simulink model "dual_thyristor_bridge_rectifier"  (R2025b)
settings: Solver=ode1be  StartTime=0.0  StopTime=simlength  FixedStep=tc  MaxStep=tc
values from neighbouring files (symbols this model uses):
  n1 = 35    [voltage_spectrum_analysis.m]
  omega_grid_emulator_nom = w_grid    (= 314.159265359)    [grid_emulator.m]
  vn_eta_pu = 0    [grid_emulator.m]
  vn_xi_pu = 0    [grid_emulator.m]
  vp_xi_pu = 1    [grid_emulator.m]
  w_grid = f_grid*2*pi    (= 314.159265359)    [grid_emulator.m]
undefined symbols (not defined in the file or in its folder): CSF_11, CSF_13, CSF_5, CSF_7, delta_fht1, Idc_traction_normalization_factor, ki_u_ctrl, kp_u_ctrl, Ld_fht1, LFu_dc, LSF_11, LSF_13, LSF_5, LSF_7, magnitude, n10, omega_fht1, pll_i1, pll_p, RLFu_dc, tc, Tcontrol_rect, ts_ctrl_rect, ugrid_factor, Vdc_traction_normalization_factor, Vgrid_phase_normalization_factor
libraries: fl_lib x299, nesl_utility x67, ee_lib x24, single_phase_transformer_lib x3, cstblocks x3
(part 3 of 6)

== system dual_thyristor_bridge_rectifier/dual_rectifier_bridge/neg_bridge/firing2 ==
  Capacitor1 : fl_lib/Electrical/Electrical Elements/Capacitor  Commented=on  c=100e-6 F  r=1e-6 Ohm  g=0 1/Ohm  i_specify=off  i_priority=None  i=0 A  i_nominal_specify=off  i_nominal_value=1  i_nominal_unit=A  v_specify=off  v_priority=None  v=0 V  v_nominal_specify=off  v_nominal_value=1  v_nominal_unit=V  vc_specify=off  vc_priority=High  vc=0 V  vc_nominal_specify=off  vc_nominal_value=1  vc_nominal_unit=V
  Capacitor2 : fl_lib/Electrical/Electrical Elements/Capacitor  Commented=on  c=100e-12 F  r=1e-6 Ohm  g=0 1/Ohm  i_specify=off  i_priority=None  i=0 A  i_nominal_specify=off  i_nominal_value=1  i_nominal_unit=A  v_specify=off  v_priority=None  v=0 V  v_nominal_specify=off  v_nominal_value=1  v_nominal_unit=V  vc_specify=off  vc_priority=High  vc=0 V  vc_nominal_specify=off  vc_nominal_value=1  vc_nominal_unit=V
  Controlled Voltage Source1 : fl_lib/Electrical/Electrical Sources/Controlled Voltage Source  Commented=on
  Controlled Voltage Source2 : fl_lib/Electrical/Electrical Sources/Controlled Voltage Source  Commented=on
  Diode : fl_lib/Electrical/Electrical Elements/Diode  Commented=on  Vf=0.6 V  Ron=0.3 Ohm  Goff=1e-8 1/Ohm  i_specify=off  i_priority=None  i=0 A  i_nominal_specify=off  i_nominal_value=1  i_nominal_unit=A  v_specify=off  v_priority=None  v=0 V  v_nominal_specify=off  v_nominal_value=1  v_nominal_unit=V
  Diode2 : fl_lib/Electrical/Electrical Elements/Diode  Commented=on  Vf=0.6 V  Ron=0.3 Ohm  Goff=1e-8 1/Ohm  i_specify=off  i_priority=None  i=0 A  i_nominal_specify=off  i_nominal_value=1  i_nominal_unit=A  v_specify=off  v_priority=None  v=0 V  v_nominal_specify=off  v_nominal_value=1  v_nominal_unit=V
  Diode3 : fl_lib/Electrical/Electrical Elements/Diode  Commented=on  Vf=0.6 V  Ron=0.3 Ohm  Goff=1e-8 1/Ohm  i_specify=off  i_priority=None  i=0 A  i_nominal_specify=off  i_nominal_value=1  i_nominal_unit=A  v_specify=off  v_priority=None  v=0 V  v_nominal_specify=off  v_nominal_value=1  v_nominal_unit=V
  Electrical Reference3 : fl_lib/Electrical/Electrical Elements/Electrical Reference  Commented=on
  Electrical Reference4 : fl_lib/Electrical/Electrical Elements/Electrical Reference  Commented=on
  Electrical Reference5 : fl_lib/Electrical/Electrical Elements/Electrical Reference  Commented=on
  "IGBT (Ideal, Switching)" : ee_lib/Semiconductors & Converters/IGBT (Ideal, Switching)  Commented=on  port_option=ee.enum.controlport.elec  Vf=0.8 V  Ron=0.001 Ohm  Goff=1e-5 1/Ohm  Vth=2 V  diode_param=1  diode_Vf=0.8 V  diode_Ron=0.001 Ohm  diode_Goff=1e-5 1/Ohm  diode_C=50e-9 F  diode_iRM=-235 A  diode_iF=300 A  diode_idot=-50 A/us  diode_trr_param=1  diode_trr_factor=3  diode_trr=15 us  diode_Qrr=1500 s*uA  ice_specify=off  ice_priority=None  ice=0 A  ice_nominal_specify=off  ice_nominal_value=1  ice_nominal_unit=A  vce_specify=off  vce_priority=None  vce=0 V  vce_nominal_specify=off  vce_nominal_value=1  vce_nominal_unit=V  vge_specify=off  vge_priority=None  vge=0 V  vge_nominal_specify=off  vge_nominal_value=1  vge_nominal_unit=V  thermal_loss_option=2  Von_data=[0, 1.1, 1.3, 1.45, 1.75, 2.25, 2.7; 0, 1, 1.15, 1.35, 1.7, 2.35, 3] V  Tj=[298.15, 398.15] K  Iout_data=[0, 10, 50, 100, 200, 400, 600] A  Eon_data=[0, .29, 1.43, 2.86, 5.71, 13.14, 22.86; 0, .57, 2.63, 5.14, 10.29, 20.57, 30.29] * 1e-3 J  Eoff_data=[0, .21, 1.07, 2.14, 4.29, 9.86, 17.14; 0, .43, 1.97, 3.86, 7.71, 15.43, 22.71] * 1e-3 J  Eon_data_3D=[zeros(2, 9, 3)] J  Eoff_data_3D=[zeros(2, 9, 3)] J  Tj_loss=[298.15, 398.15] K  Iout_data_loss=[0, .1, 1, 5, 10, 20, 40, 70, 100] A  tabulateWithVce=false  Vce_loss=[0, 150, 300] V  Eon_scalar=22.86e-3 J  Eoff_scalar=17.14e-3 J  Voff=300 V  Iout_scalar=600 A  useCurrentFromPreviousCycle=false  useVoltageFromPreviousCycle=false  diodeModelType=ee.enum.converters.diodeModelType.pwl  diodeTableType=ee.enum.diode.tableType.IfMat  diode_ReverseIVType=ee.enum.diode.diodeReverseIV.constant  diode_IfMat=[.07, .12, .19, 1.75, 4.24, 7.32, 11.2; .16, .3, .72, 2.14, 4.02, 6.35, 9.12] A  diode_VfMat=[.9, 1.15, 1.25, 1.5, 1.75, 2.17, 2.6, 2.85; .58, .68, .75, 1.1, 1.38, 1.77, 2.27, 2.7] V  diode_TjVec=[25, 125] degC  diode_VfVec=[.5, .7, .9, 1.3, 1.7, 2.1, 2.5] V  diode_IfVec=[.1, .2, .5, 1, 2, 4, 7, 10] A  diode_IrMat=[1e-06, 2e-06, 5e-06, 1e-05, 2.5e-05, 5e-05, .0001; 2e-06, 5e-06, 1e-05, 4e-05, 8e-05, .0002, .0005] A  diode_VrMat=[10, 100, 200, 250, 300, 325, 350; 10, 70, 160, 220, 270, 300, 320] V  diode_VrVec=[10, 20, 40, 50, 70, 80, 100] V  diode_IrVec=[1e-06, 2e-06, 5e-06, 1e-05, 2e-05, 5e-05, .0001] A  diode_Vr=-600 V  diode_Ls=150 nH  diode_Erec=0.03 J  diode_rec_loss_model=ee.enum.diode.reverseRecoveryModel.fixed  diode_ErecVal=0 J  diode_scaleWithIandV=true  diode_ErecMat=zeros(2, 3) J  diode_TjrecVec=[298.15, 398.15] K  diode_IfrecVec=[.1, 1, 10] A  diode_IrecVal=10 A  diode_VrecVal=10 V  diode_tFilter=1 / 1000 / 100 s  separateThermalPortForDiode=false  thermal_network_parameterization=ee.enum.thermalNetworkTopology.external  Rth=[.08, .5] K/W  Rth_Cauer=[.08, .1, .5] K/W  Rth_Foster=[.08, .14, .22, .16] K/W  thermal_mass_parameterization=ee.enum.thermalNetwork.timeconstant  thermal_mass=[.01, .5] J/K  thermal_mass_Cauer=[.01, .1, .5] J/K  thermal_mass_Foster=[.001, .005, .05, .5] J/K  thermal_time_constant=[.001, .2] s  thermal_time_constant_Cauer=[.001, .1, .2] s  thermal_time_constant_Foster=[7e-05, .0007, .01, .08] s  thermal_mass_initial_temperatures=[25, 25] degC  thermal_mass_initial_temperatures_Cauer=[25, 25, 25] degC  junction_thermal_mass=0.01 J/K  Tvec_initial_Foster=[25, 25, 25, 25] degC  RthDiode=[.03, .2] K/W  RthCauerDiode=[.03, .1, .2] K/W  RthFosterDiode=[.03, .2] K/W  thermalMassDiode=[3, 25] J/K  thermalMassCauerDiode=[3, 10, 25] J/K  thermalMassFosterDiode=[33, 50] J/K  thermalTauDiode=[.1, 5] s  thermalTauCauerDiode=[.1, 1, 5] s  thermalTauFosterDiode=[1, 10] s  thermalMassInitTempDiode=[25, 25] degC  thermalMassInitTempCauerDiode=[25, 25, 25] degC  junctionthermalMassDiode=0.1 J/K  TVecInitialFosterDiode=[25, 25, 25, 25] degC  no_thermal_network=0  IGBT_junction_temperature_specify=off  IGBT_junction_temperature_priority=None  IGBT_junction_temperature=25 degC  IGBT_junction_temperature_nominal_specify=off  IGBT_junction_temperature_nominal_value=1  IGBT_junction_temperature_nominal_unit=degC  diode_junction_temperature_specify=off  diode_junction_temperature_priority=None  diode_junction_temperature=25 degC  diode_junction_temperature_nominal_specify=off  diode_junction_temperature_nominal_value=1  diode_junction_temperature_nominal_unit=degC  Qj_specify=off  Qj_priority=None  Qj=0 W  Qj_nominal_specify=off  Qj_nominal_value=1  Qj_nominal_unit=W  accumulatedSwitchingLosses_specify=off  accumulatedSwitchingLosses_priority=None  accumulatedSwitchingLosses=0 J
      settings: InternalSimscapePortConfiguration="{\"Bottom\":[],\"Left\":[{\"id\":\"G_elec\",\"label\":\"\",\"type\":\"foundation.electrical.electrical\"}],\"Right\":[{\"id\":\"C\",\"label\":\"\",\"type\":\"foundation.electrical.electrical\"},{\"id\":\"E\",\"label\":\"\",\"type\":\"foundation.electrical.electrical\"}],\"Top\":[]}"
  Ideal Transformer : fl_lib/Electrical/Electrical Elements/Ideal Transformer  Commented=on  n=2  i1_specify=off  i1_priority=None  i1=0 A  i1_nominal_specify=off  i1_nominal_value=1  i1_nominal_unit=A  v1_specify=off  v1_priority=None  v1=0 V  v1_nominal_specify=off  v1_nominal_value=1  v1_nominal_unit=V  i2_specify=off  i2_priority=None  i2=0 A  i2_nominal_specify=off  i2_nominal_value=1  i2_nominal_unit=A  v2_specify=off  v2_priority=None  v2=0 V  v2_nominal_specify=off  v2_nominal_value=1  v2_nominal_unit=V
  PS Constant : fl_lib/Physical Signals/Sources/PS Constant  Commented=on  constant=48 V
  Resistor1 : fl_lib/Electrical/Electrical Elements/Resistor  Commented=on  R=470 Ohm  i_specify=off  i_priority=None  i=0 A  i_nominal_specify=off  i_nominal_value=1  i_nominal_unit=A  v_specify=off  v_priority=None  v=0 V  v_nominal_specify=off  v_nominal_value=1  v_nominal_unit=V
  Resistor3 : fl_lib/Electrical/Electrical Elements/Resistor  Commented=on  R=470 Ohm  i_specify=off  i_priority=None  i=0 A  i_nominal_specify=off  i_nominal_value=1  i_nominal_unit=A  v_specify=off  v_priority=None  v=0 V  v_nominal_specify=off  v_nominal_value=1  v_nominal_unit=V
  Resistor5 : fl_lib/Electrical/Electrical Elements/Resistor  Commented=on  R=100 Ohm  i_specify=off  i_priority=None  i=0 A  i_nominal_specify=off  i_nominal_value=1  i_nominal_unit=A  v_specify=off  v_priority=None  v=0 V  v_nominal_specify=off  v_nominal_value=1  v_nominal_unit=V
  Resistor6 : fl_lib/Electrical/Electrical Elements/Resistor  Commented=on  R=1e9 Ohm  i_specify=off  i_priority=None  i=0 A  i_nominal_specify=off  i_nominal_value=1  i_nominal_unit=A  v_specify=off  v_priority=None  v=0 V  v_nominal_specify=off  v_nominal_value=1  v_nominal_unit=V
  Voltage Sensor : fl_lib/Electrical/Electrical Sensors/Voltage Sensor  Commented=on
  oscillator : Subsystem  Commented=on
  gin : PMIOPort  Side=Left
  g+ : PMIOPort  Port=2  Side=Right
  connections:
  "IGBT (Ideal, Switching)"/LConn1 -- Resistor1/RConn1
  Electrical Reference4/LConn1 -- Diode/LConn1 -- Ideal Transformer/LConn2
  Controlled Voltage Source2/LConn1 -- Resistor1/LConn1
  Controlled Voltage Source2/RConn2 -- Controlled Voltage Source1/RConn2 -- "IGBT (Ideal, Switching)"/RConn2 -- Ideal Transformer/LConn1 -- Diode/RConn1
  Ideal Transformer/RConn1 -- Diode2/LConn1
  Capacitor2/RConn1 -- Voltage Sensor/RConn2 -- Ideal Transformer/RConn2 -- Resistor6/LConn1 -- Resistor5/RConn1
  Diode2/RConn1 -- Resistor5/LConn1 -- Voltage Sensor/LConn1 -- Capacitor2/LConn1
  PS Constant/RConn1 -- Controlled Voltage Source1/RConn1
  Resistor6/RConn1 -- Electrical Reference3/LConn1
  "IGBT (Ideal, Switching)"/RConn1 -- Diode3/RConn1
  Diode3/LConn1 -- Resistor3/RConn1 -- Capacitor1/LConn1
  Electrical Reference5/LConn1 -- Capacitor1/RConn1
  Resistor3/LConn1 -- Controlled Voltage Source1/LConn1
  gin/RConn1 -- g+/RConn1

== system dual_thyristor_bridge_rectifier/dual_rectifier_bridge/neg_bridge/firing3 ==
  Capacitor1 : fl_lib/Electrical/Electrical Elements/Capacitor  Commented=on  c=100e-6 F  r=1e-6 Ohm  g=0 1/Ohm  i_specify=off  i_priority=None  i=0 A  i_nominal_specify=off  i_nominal_value=1  i_nominal_unit=A  v_specify=off  v_priority=None  v=0 V  v_nominal_specify=off  v_nominal_value=1  v_nominal_unit=V  vc_specify=off  vc_priority=High  vc=0 V  vc_nominal_specify=off  vc_nominal_value=1  vc_nominal_unit=V
  Capacitor2 : fl_lib/Electrical/Electrical Elements/Capacitor  Commented=on  c=100e-12 F  r=1e-6 Ohm  g=0 1/Ohm  i_specify=off  i_priority=None  i=0 A  i_nominal_specify=off  i_nominal_value=1  i_nominal_unit=A  v_specify=off  v_priority=None  v=0 V  v_nominal_specify=off  v_nominal_value=1  v_nominal_unit=V  vc_specify=off  vc_priority=High  vc=0 V  vc_nominal_specify=off  vc_nominal_value=1  vc_nominal_unit=V
  Controlled Voltage Source1 : fl_lib/Electrical/Electrical Sources/Controlled Voltage Source  Commented=on
  Controlled Voltage Source2 : fl_lib/Electrical/Electrical Sources/Controlled Voltage Source  Commented=on
  Diode : fl_lib/Electrical/Electrical Elements/Diode  Commented=on  Vf=0.6 V  Ron=0.3 Ohm  Goff=1e-8 1/Ohm  i_specify=off  i_priority=None  i=0 A  i_nominal_specify=off  i_nominal_value=1  i_nominal_unit=A  v_specify=off  v_priority=None  v=0 V  v_nominal_specify=off  v_nominal_value=1  v_nominal_unit=V
  Diode2 : fl_lib/Electrical/Electrical Elements/Diode  Commented=on  Vf=0.6 V  Ron=0.3 Ohm  Goff=1e-8 1/Ohm  i_specify=off  i_priority=None  i=0 A  i_nominal_specify=off  i_nominal_value=1  i_nominal_unit=A  v_specify=off  v_priority=None  v=0 V  v_nominal_specify=off  v_nominal_value=1  v_nominal_unit=V
  Diode3 : fl_lib/Electrical/Electrical Elements/Diode  Commented=on  Vf=0.6 V  Ron=0.3 Ohm  Goff=1e-8 1/Ohm  i_specify=off  i_priority=None  i=0 A  i_nominal_specify=off  i_nominal_value=1  i_nominal_unit=A  v_specify=off  v_priority=None  v=0 V  v_nominal_specify=off  v_nominal_value=1  v_nominal_unit=V
  Electrical Reference3 : fl_lib/Electrical/Electrical Elements/Electrical Reference  Commented=on
  Electrical Reference4 : fl_lib/Electrical/Electrical Elements/Electrical Reference  Commented=on
  Electrical Reference5 : fl_lib/Electrical/Electrical Elements/Electrical Reference  Commented=on
  "IGBT (Ideal, Switching)" : ee_lib/Semiconductors & Converters/IGBT (Ideal, Switching)  Commented=on  port_option=ee.enum.controlport.elec  Vf=0.8 V  Ron=0.001 Ohm  Goff=1e-5 1/Ohm  Vth=2 V  diode_param=1  diode_Vf=0.8 V  diode_Ron=0.001 Ohm  diode_Goff=1e-5 1/Ohm  diode_C=50e-9 F  diode_iRM=-235 A  diode_iF=300 A  diode_idot=-50 A/us  diode_trr_param=1  diode_trr_factor=3  diode_trr=15 us  diode_Qrr=1500 s*uA  ice_specify=off  ice_priority=None  ice=0 A  ice_nominal_specify=off  ice_nominal_value=1  ice_nominal_unit=A  vce_specify=off  vce_priority=None  vce=0 V  vce_nominal_specify=off  vce_nominal_value=1  vce_nominal_unit=V  vge_specify=off  vge_priority=None  vge=0 V  vge_nominal_specify=off  vge_nominal_value=1  vge_nominal_unit=V  thermal_loss_option=2  Von_data=[0, 1.1, 1.3, 1.45, 1.75, 2.25, 2.7; 0, 1, 1.15, 1.35, 1.7, 2.35, 3] V  Tj=[298.15, 398.15] K  Iout_data=[0, 10, 50, 100, 200, 400, 600] A  Eon_data=[0, .29, 1.43, 2.86, 5.71, 13.14, 22.86; 0, .57, 2.63, 5.14, 10.29, 20.57, 30.29] * 1e-3 J  Eoff_data=[0, .21, 1.07, 2.14, 4.29, 9.86, 17.14; 0, .43, 1.97, 3.86, 7.71, 15.43, 22.71] * 1e-3 J  Eon_data_3D=[zeros(2, 9, 3)] J  Eoff_data_3D=[zeros(2, 9, 3)] J  Tj_loss=[298.15, 398.15] K  Iout_data_loss=[0, .1, 1, 5, 10, 20, 40, 70, 100] A  tabulateWithVce=false  Vce_loss=[0, 150, 300] V  Eon_scalar=22.86e-3 J  Eoff_scalar=17.14e-3 J  Voff=300 V  Iout_scalar=600 A  useCurrentFromPreviousCycle=false  useVoltageFromPreviousCycle=false  diodeModelType=ee.enum.converters.diodeModelType.pwl  diodeTableType=ee.enum.diode.tableType.IfMat  diode_ReverseIVType=ee.enum.diode.diodeReverseIV.constant  diode_IfMat=[.07, .12, .19, 1.75, 4.24, 7.32, 11.2; .16, .3, .72, 2.14, 4.02, 6.35, 9.12] A  diode_VfMat=[.9, 1.15, 1.25, 1.5, 1.75, 2.17, 2.6, 2.85; .58, .68, .75, 1.1, 1.38, 1.77, 2.27, 2.7] V  diode_TjVec=[25, 125] degC  diode_VfVec=[.5, .7, .9, 1.3, 1.7, 2.1, 2.5] V  diode_IfVec=[.1, .2, .5, 1, 2, 4, 7, 10] A  diode_IrMat=[1e-06, 2e-06, 5e-06, 1e-05, 2.5e-05, 5e-05, .0001; 2e-06, 5e-06, 1e-05, 4e-05, 8e-05, .0002, .0005] A  diode_VrMat=[10, 100, 200, 250, 300, 325, 350; 10, 70, 160, 220, 270, 300, 320] V  diode_VrVec=[10, 20, 40, 50, 70, 80, 100] V  diode_IrVec=[1e-06, 2e-06, 5e-06, 1e-05, 2e-05, 5e-05, .0001] A  diode_Vr=-600 V  diode_Ls=150 nH  diode_Erec=0.03 J  diode_rec_loss_model=ee.enum.diode.reverseRecoveryModel.fixed  diode_ErecVal=0 J  diode_scaleWithIandV=true  diode_ErecMat=zeros(2, 3) J  diode_TjrecVec=[298.15, 398.15] K  diode_IfrecVec=[.1, 1, 10] A  diode_IrecVal=10 A  diode_VrecVal=10 V  diode_tFilter=1 / 1000 / 100 s  separateThermalPortForDiode=false  thermal_network_parameterization=ee.enum.thermalNetworkTopology.external  Rth=[.08, .5] K/W  Rth_Cauer=[.08, .1, .5] K/W  Rth_Foster=[.08, .14, .22, .16] K/W  thermal_mass_parameterization=ee.enum.thermalNetwork.timeconstant  thermal_mass=[.01, .5] J/K  thermal_mass_Cauer=[.01, .1, .5] J/K  thermal_mass_Foster=[.001, .005, .05, .5] J/K  thermal_time_constant=[.001, .2] s  thermal_time_constant_Cauer=[.001, .1, .2] s  thermal_time_constant_Foster=[7e-05, .0007, .01, .08] s  thermal_mass_initial_temperatures=[25, 25] degC  thermal_mass_initial_temperatures_Cauer=[25, 25, 25] degC  junction_thermal_mass=0.01 J/K  Tvec_initial_Foster=[25, 25, 25, 25] degC  RthDiode=[.03, .2] K/W  RthCauerDiode=[.03, .1, .2] K/W  RthFosterDiode=[.03, .2] K/W  thermalMassDiode=[3, 25] J/K  thermalMassCauerDiode=[3, 10, 25] J/K  thermalMassFosterDiode=[33, 50] J/K  thermalTauDiode=[.1, 5] s  thermalTauCauerDiode=[.1, 1, 5] s  thermalTauFosterDiode=[1, 10] s  thermalMassInitTempDiode=[25, 25] degC  thermalMassInitTempCauerDiode=[25, 25, 25] degC  junctionthermalMassDiode=0.1 J/K  TVecInitialFosterDiode=[25, 25, 25, 25] degC  no_thermal_network=0  IGBT_junction_temperature_specify=off  IGBT_junction_temperature_priority=None  IGBT_junction_temperature=25 degC  IGBT_junction_temperature_nominal_specify=off  IGBT_junction_temperature_nominal_value=1  IGBT_junction_temperature_nominal_unit=degC  diode_junction_temperature_specify=off  diode_junction_temperature_priority=None  diode_junction_temperature=25 degC  diode_junction_temperature_nominal_specify=off  diode_junction_temperature_nominal_value=1  diode_junction_temperature_nominal_unit=degC  Qj_specify=off  Qj_priority=None  Qj=0 W  Qj_nominal_specify=off  Qj_nominal_value=1  Qj_nominal_unit=W  accumulatedSwitchingLosses_specify=off  accumulatedSwitchingLosses_priority=None  accumulatedSwitchingLosses=0 J
      settings: InternalSimscapePortConfiguration="{\"Bottom\":[],\"Left\":[{\"id\":\"G_elec\",\"label\":\"\",\"type\":\"foundation.electrical.electrical\"}],\"Right\":[{\"id\":\"C\",\"label\":\"\",\"type\":\"foundation.electrical.electrical\"},{\"id\":\"E\",\"label\":\"\",\"type\":\"foundation.electrical.electrical\"}],\"Top\":[]}"
  Ideal Transformer : fl_lib/Electrical/Electrical Elements/Ideal Transformer  Commented=on  n=2  i1_specify=off  i1_priority=None  i1=0 A  i1_nominal_specify=off  i1_nominal_value=1  i1_nominal_unit=A  v1_specify=off  v1_priority=None  v1=0 V  v1_nominal_specify=off  v1_nominal_value=1  v1_nominal_unit=V  i2_specify=off  i2_priority=None  i2=0 A  i2_nominal_specify=off  i2_nominal_value=1  i2_nominal_unit=A  v2_specify=off  v2_priority=None  v2=0 V  v2_nominal_specify=off  v2_nominal_value=1  v2_nominal_unit=V
  PS Constant : fl_lib/Physical Signals/Sources/PS Constant  Commented=on  constant=48 V
  Resistor1 : fl_lib/Electrical/Electrical Elements/Resistor  Commented=on  R=470 Ohm  i_specify=off  i_priority=None  i=0 A  i_nominal_specify=off  i_nominal_value=1  i_nominal_unit=A  v_specify=off  v_priority=None  v=0 V  v_nominal_specify=off  v_nominal_value=1  v_nominal_unit=V
  Resistor3 : fl_lib/Electrical/Electrical Elements/Resistor  Commented=on  R=470 Ohm  i_specify=off  i_priority=None  i=0 A  i_nominal_specify=off  i_nominal_value=1  i_nominal_unit=A  v_specify=off  v_priority=None  v=0 V  v_nominal_specify=off  v_nominal_value=1  v_nominal_unit=V
  Resistor5 : fl_lib/Electrical/Electrical Elements/Resistor  Commented=on  R=100 Ohm  i_specify=off  i_priority=None  i=0 A  i_nominal_specify=off  i_nominal_value=1  i_nominal_unit=A  v_specify=off  v_priority=None  v=0 V  v_nominal_specify=off  v_nominal_value=1  v_nominal_unit=V
  Resistor6 : fl_lib/Electrical/Electrical Elements/Resistor  Commented=on  R=1e9 Ohm  i_specify=off  i_priority=None  i=0 A  i_nominal_specify=off  i_nominal_value=1  i_nominal_unit=A  v_specify=off  v_priority=None  v=0 V  v_nominal_specify=off  v_nominal_value=1  v_nominal_unit=V
  Voltage Sensor : fl_lib/Electrical/Electrical Sensors/Voltage Sensor  Commented=on
  oscillator : Subsystem  Commented=on
  gin : PMIOPort  Side=Left
  g+ : PMIOPort  Port=2  Side=Right
  connections:
  Resistor3/LConn1 -- Controlled Voltage Source1/LConn1
  Electrical Reference5/LConn1 -- Capacitor1/RConn1
  Capacitor1/LConn1 -- Resistor3/RConn1 -- Diode3/LConn1
  "IGBT (Ideal, Switching)"/RConn1 -- Diode3/RConn1
  Resistor6/RConn1 -- Electrical Reference3/LConn1
  PS Constant/RConn1 -- Controlled Voltage Source1/RConn1
  Capacitor2/LConn1 -- Voltage Sensor/LConn1 -- Resistor5/LConn1 -- Diode2/RConn1
  Resistor5/RConn1 -- Resistor6/LConn1 -- Ideal Transformer/RConn2 -- Voltage Sensor/RConn2 -- Capacitor2/RConn1
  Ideal Transformer/RConn1 -- Diode2/LConn1
  Diode/RConn1 -- Ideal Transformer/LConn1 -- "IGBT (Ideal, Switching)"/RConn2 -- Controlled Voltage Source1/RConn2 -- Controlled Voltage Source2/RConn2
  Controlled Voltage Source2/LConn1 -- Resistor1/LConn1
  Ideal Transformer/LConn2 -- Diode/LConn1 -- Electrical Reference4/LConn1
  "IGBT (Ideal, Switching)"/LConn1 -- Resistor1/RConn1
  gin/RConn1 -- g+/RConn1

== system dual_thyristor_bridge_rectifier/dual_rectifier_bridge/neg_bridge/firing4 ==
  Capacitor1 : fl_lib/Electrical/Electrical Elements/Capacitor  Commented=on  c=100e-6 F  r=1e-6 Ohm  g=0 1/Ohm  i_specify=off  i_priority=None  i=0 A  i_nominal_specify=off  i_nominal_value=1  i_nominal_unit=A  v_specify=off  v_priority=None  v=0 V  v_nominal_specify=off  v_nominal_value=1  v_nominal_unit=V  vc_specify=off  vc_priority=High  vc=0 V  vc_nominal_specify=off  vc_nominal_value=1  vc_nominal_unit=V
  Capacitor2 : fl_lib/Electrical/Electrical Elements/Capacitor  Commented=on  c=100e-12 F  r=1e-6 Ohm  g=0 1/Ohm  i_specify=off  i_priority=None  i=0 A  i_nominal_specify=off  i_nominal_value=1  i_nominal_unit=A  v_specify=off  v_priority=None  v=0 V  v_nominal_specify=off  v_nominal_value=1  v_nominal_unit=V  vc_specify=off  vc_priority=High  vc=0 V  vc_nominal_specify=off  vc_nominal_value=1  vc_nominal_unit=V
  Controlled Voltage Source1 : fl_lib/Electrical/Electrical Sources/Controlled Voltage Source  Commented=on
  Controlled Voltage Source2 : fl_lib/Electrical/Electrical Sources/Controlled Voltage Source  Commented=on
  Diode : fl_lib/Electrical/Electrical Elements/Diode  Commented=on  Vf=0.6 V  Ron=0.3 Ohm  Goff=1e-8 1/Ohm  i_specify=off  i_priority=None  i=0 A  i_nominal_specify=off  i_nominal_value=1  i_nominal_unit=A  v_specify=off  v_priority=None  v=0 V  v_nominal_specify=off  v_nominal_value=1  v_nominal_unit=V
  Diode2 : fl_lib/Electrical/Electrical Elements/Diode  Commented=on  Vf=0.6 V  Ron=0.3 Ohm  Goff=1e-8 1/Ohm  i_specify=off  i_priority=None  i=0 A  i_nominal_specify=off  i_nominal_value=1  i_nominal_unit=A  v_specify=off  v_priority=None  v=0 V  v_nominal_specify=off  v_nominal_value=1  v_nominal_unit=V
  Diode3 : fl_lib/Electrical/Electrical Elements/Diode  Commented=on  Vf=0.6 V  Ron=0.3 Ohm  Goff=1e-8 1/Ohm  i_specify=off  i_priority=None  i=0 A  i_nominal_specify=off  i_nominal_value=1  i_nominal_unit=A  v_specify=off  v_priority=None  v=0 V  v_nominal_specify=off  v_nominal_value=1  v_nominal_unit=V
  Electrical Reference3 : fl_lib/Electrical/Electrical Elements/Electrical Reference  Commented=on
  Electrical Reference4 : fl_lib/Electrical/Electrical Elements/Electrical Reference  Commented=on
  Electrical Reference5 : fl_lib/Electrical/Electrical Elements/Electrical Reference  Commented=on
  "IGBT (Ideal, Switching)" : ee_lib/Semiconductors & Converters/IGBT (Ideal, Switching)  Commented=on  port_option=ee.enum.controlport.elec  Vf=0.8 V  Ron=0.001 Ohm  Goff=1e-5 1/Ohm  Vth=2 V  diode_param=1  diode_Vf=0.8 V  diode_Ron=0.001 Ohm  diode_Goff=1e-5 1/Ohm  diode_C=50e-9 F  diode_iRM=-235 A  diode_iF=300 A  diode_idot=-50 A/us  diode_trr_param=1  diode_trr_factor=3  diode_trr=15 us  diode_Qrr=1500 s*uA  ice_specify=off  ice_priority=None  ice=0 A  ice_nominal_specify=off  ice_nominal_value=1  ice_nominal_unit=A  vce_specify=off  vce_priority=None  vce=0 V  vce_nominal_specify=off  vce_nominal_value=1  vce_nominal_unit=V  vge_specify=off  vge_priority=None  vge=0 V  vge_nominal_specify=off  vge_nominal_value=1  vge_nominal_unit=V  thermal_loss_option=2  Von_data=[0, 1.1, 1.3, 1.45, 1.75, 2.25, 2.7; 0, 1, 1.15, 1.35, 1.7, 2.35, 3] V  Tj=[298.15, 398.15] K  Iout_data=[0, 10, 50, 100, 200, 400, 600] A  Eon_data=[0, .29, 1.43, 2.86, 5.71, 13.14, 22.86; 0, .57, 2.63, 5.14, 10.29, 20.57, 30.29] * 1e-3 J  Eoff_data=[0, .21, 1.07, 2.14, 4.29, 9.86, 17.14; 0, .43, 1.97, 3.86, 7.71, 15.43, 22.71] * 1e-3 J  Eon_data_3D=[zeros(2, 9, 3)] J  Eoff_data_3D=[zeros(2, 9, 3)] J  Tj_loss=[298.15, 398.15] K  Iout_data_loss=[0, .1, 1, 5, 10, 20, 40, 70, 100] A  tabulateWithVce=false  Vce_loss=[0, 150, 300] V  Eon_scalar=22.86e-3 J  Eoff_scalar=17.14e-3 J  Voff=300 V  Iout_scalar=600 A  useCurrentFromPreviousCycle=false  useVoltageFromPreviousCycle=false  diodeModelType=ee.enum.converters.diodeModelType.pwl  diodeTableType=ee.enum.diode.tableType.IfMat  diode_ReverseIVType=ee.enum.diode.diodeReverseIV.constant  diode_IfMat=[.07, .12, .19, 1.75, 4.24, 7.32, 11.2; .16, .3, .72, 2.14, 4.02, 6.35, 9.12] A  diode_VfMat=[.9, 1.15, 1.25, 1.5, 1.75, 2.17, 2.6, 2.85; .58, .68, .75, 1.1, 1.38, 1.77, 2.27, 2.7] V  diode_TjVec=[25, 125] degC  diode_VfVec=[.5, .7, .9, 1.3, 1.7, 2.1, 2.5] V  diode_IfVec=[.1, .2, .5, 1, 2, 4, 7, 10] A  diode_IrMat=[1e-06, 2e-06, 5e-06, 1e-05, 2.5e-05, 5e-05, .0001; 2e-06, 5e-06, 1e-05, 4e-05, 8e-05, .0002, .0005] A  diode_VrMat=[10, 100, 200, 250, 300, 325, 350; 10, 70, 160, 220, 270, 300, 320] V  diode_VrVec=[10, 20, 40, 50, 70, 80, 100] V  diode_IrVec=[1e-06, 2e-06, 5e-06, 1e-05, 2e-05, 5e-05, .0001] A  diode_Vr=-600 V  diode_Ls=150 nH  diode_Erec=0.03 J  diode_rec_loss_model=ee.enum.diode.reverseRecoveryModel.fixed  diode_ErecVal=0 J  diode_scaleWithIandV=true  diode_ErecMat=zeros(2, 3) J  diode_TjrecVec=[298.15, 398.15] K  diode_IfrecVec=[.1, 1, 10] A  diode_IrecVal=10 A  diode_VrecVal=10 V  diode_tFilter=1 / 1000 / 100 s  separateThermalPortForDiode=false  thermal_network_parameterization=ee.enum.thermalNetworkTopology.external  Rth=[.08, .5] K/W  Rth_Cauer=[.08, .1, .5] K/W  Rth_Foster=[.08, .14, .22, .16] K/W  thermal_mass_parameterization=ee.enum.thermalNetwork.timeconstant  thermal_mass=[.01, .5] J/K  thermal_mass_Cauer=[.01, .1, .5] J/K  thermal_mass_Foster=[.001, .005, .05, .5] J/K  thermal_time_constant=[.001, .2] s  thermal_time_constant_Cauer=[.001, .1, .2] s  thermal_time_constant_Foster=[7e-05, .0007, .01, .08] s  thermal_mass_initial_temperatures=[25, 25] degC  thermal_mass_initial_temperatures_Cauer=[25, 25, 25] degC  junction_thermal_mass=0.01 J/K  Tvec_initial_Foster=[25, 25, 25, 25] degC  RthDiode=[.03, .2] K/W  RthCauerDiode=[.03, .1, .2] K/W  RthFosterDiode=[.03, .2] K/W  thermalMassDiode=[3, 25] J/K  thermalMassCauerDiode=[3, 10, 25] J/K  thermalMassFosterDiode=[33, 50] J/K  thermalTauDiode=[.1, 5] s  thermalTauCauerDiode=[.1, 1, 5] s  thermalTauFosterDiode=[1, 10] s  thermalMassInitTempDiode=[25, 25] degC  thermalMassInitTempCauerDiode=[25, 25, 25] degC  junctionthermalMassDiode=0.1 J/K  TVecInitialFosterDiode=[25, 25, 25, 25] degC  no_thermal_network=0  IGBT_junction_temperature_specify=off  IGBT_junction_temperature_priority=None  IGBT_junction_temperature=25 degC  IGBT_junction_temperature_nominal_specify=off  IGBT_junction_temperature_nominal_value=1  IGBT_junction_temperature_nominal_unit=degC  diode_junction_temperature_specify=off  diode_junction_temperature_priority=None  diode_junction_temperature=25 degC  diode_junction_temperature_nominal_specify=off  diode_junction_temperature_nominal_value=1  diode_junction_temperature_nominal_unit=degC  Qj_specify=off  Qj_priority=None  Qj=0 W  Qj_nominal_specify=off  Qj_nominal_value=1  Qj_nominal_unit=W  accumulatedSwitchingLosses_specify=off  accumulatedSwitchingLosses_priority=None  accumulatedSwitchingLosses=0 J
      settings: InternalSimscapePortConfiguration="{\"Bottom\":[],\"Left\":[{\"id\":\"G_elec\",\"label\":\"\",\"type\":\"foundation.electrical.electrical\"}],\"Right\":[{\"id\":\"C\",\"label\":\"\",\"type\":\"foundation.electrical.electrical\"},{\"id\":\"E\",\"label\":\"\",\"type\":\"foundation.electrical.electrical\"}],\"Top\":[]}"
  Ideal Transformer : fl_lib/Electrical/Electrical Elements/Ideal Transformer  Commented=on  n=2  i1_specify=off  i1_priority=None  i1=0 A  i1_nominal_specify=off  i1_nominal_value=1  i1_nominal_unit=A  v1_specify=off  v1_priority=None  v1=0 V  v1_nominal_specify=off  v1_nominal_value=1  v1_nominal_unit=V  i2_specify=off  i2_priority=None  i2=0 A  i2_nominal_specify=off  i2_nominal_value=1  i2_nominal_unit=A  v2_specify=off  v2_priority=None  v2=0 V  v2_nominal_specify=off  v2_nominal_value=1  v2_nominal_unit=V
  PS Constant : fl_lib/Physical Signals/Sources/PS Constant  Commented=on  constant=48 V
  Resistor1 : fl_lib/Electrical/Electrical Elements/Resistor  Commented=on  R=470 Ohm  i_specify=off  i_priority=None  i=0 A  i_nominal_specify=off  i_nominal_value=1  i_nominal_unit=A  v_specify=off  v_priority=None  v=0 V  v_nominal_specify=off  v_nominal_value=1  v_nominal_unit=V
  Resistor3 : fl_lib/Electrical/Electrical Elements/Resistor  Commented=on  R=470 Ohm  i_specify=off  i_priority=None  i=0 A  i_nominal_specify=off  i_nominal_value=1  i_nominal_unit=A  v_specify=off  v_priority=None  v=0 V  v_nominal_specify=off  v_nominal_value=1  v_nominal_unit=V
  Resistor5 : fl_lib/Electrical/Electrical Elements/Resistor  Commented=on  R=100 Ohm  i_specify=off  i_priority=None  i=0 A  i_nominal_specify=off  i_nominal_value=1  i_nominal_unit=A  v_specify=off  v_priority=None  v=0 V  v_nominal_specify=off  v_nominal_value=1  v_nominal_unit=V
  Resistor6 : fl_lib/Electrical/Electrical Elements/Resistor  Commented=on  R=1e9 Ohm  i_specify=off  i_priority=None  i=0 A  i_nominal_specify=off  i_nominal_value=1  i_nominal_unit=A  v_specify=off  v_priority=None  v=0 V  v_nominal_specify=off  v_nominal_value=1  v_nominal_unit=V
  Voltage Sensor : fl_lib/Electrical/Electrical Sensors/Voltage Sensor  Commented=on
  oscillator : Subsystem  Commented=on
  gin : PMIOPort  Side=Left
  g+ : PMIOPort  Port=2  Side=Right
  connections:
  "IGBT (Ideal, Switching)"/LConn1 -- Resistor1/RConn1
  Electrical Reference4/LConn1 -- Diode/LConn1 -- Ideal Transformer/LConn2
  Controlled Voltage Source2/LConn1 -- Resistor1/LConn1
  Controlled Voltage Source2/RConn2 -- Controlled Voltage Source1/RConn2 -- "IGBT (Ideal, Switching)"/RConn2 -- Ideal Transformer/LConn1 -- Diode/RConn1
  Ideal Transformer/RConn1 -- Diode2/LConn1
  Capacitor2/RConn1 -- Voltage Sensor/RConn2 -- Ideal Transformer/RConn2 -- Resistor6/LConn1 -- Resistor5/RConn1
  Diode2/RConn1 -- Resistor5/LConn1 -- Voltage Sensor/LConn1 -- Capacitor2/LConn1
  PS Constant/RConn1 -- Controlled Voltage Source1/RConn1
  Resistor6/RConn1 -- Electrical Reference3/LConn1
  "IGBT (Ideal, Switching)"/RConn1 -- Diode3/RConn1
  Diode3/LConn1 -- Resistor3/RConn1 -- Capacitor1/LConn1
  Electrical Reference5/LConn1 -- Capacitor1/RConn1
  Resistor3/LConn1 -- Controlled Voltage Source1/LConn1
  gin/RConn1 -- g+/RConn1

== system dual_thyristor_bridge_rectifier/dual_rectifier_bridge/neg_bridge/firing5 ==
  Capacitor1 : fl_lib/Electrical/Electrical Elements/Capacitor  Commented=on  c=100e-6 F  r=1e-6 Ohm  g=0 1/Ohm  i_specify=off  i_priority=None  i=0 A  i_nominal_specify=off  i_nominal_value=1  i_nominal_unit=A  v_specify=off  v_priority=None  v=0 V  v_nominal_specify=off  v_nominal_value=1  v_nominal_unit=V  vc_specify=off  vc_priority=High  vc=0 V  vc_nominal_specify=off  vc_nominal_value=1  vc_nominal_unit=V
  Capacitor2 : fl_lib/Electrical/Electrical Elements/Capacitor  Commented=on  c=100e-12 F  r=1e-6 Ohm  g=0 1/Ohm  i_specify=off  i_priority=None  i=0 A  i_nominal_specify=off  i_nominal_value=1  i_nominal_unit=A  v_specify=off  v_priority=None  v=0 V  v_nominal_specify=off  v_nominal_value=1  v_nominal_unit=V  vc_specify=off  vc_priority=High  vc=0 V  vc_nominal_specify=off  vc_nominal_value=1  vc_nominal_unit=V
  Controlled Voltage Source1 : fl_lib/Electrical/Electrical Sources/Controlled Voltage Source  Commented=on
  Controlled Voltage Source2 : fl_lib/Electrical/Electrical Sources/Controlled Voltage Source  Commented=on
  Diode : fl_lib/Electrical/Electrical Elements/Diode  Commented=on  Vf=0.6 V  Ron=0.3 Ohm  Goff=1e-8 1/Ohm  i_specify=off  i_priority=None  i=0 A  i_nominal_specify=off  i_nominal_value=1  i_nominal_unit=A  v_specify=off  v_priority=None  v=0 V  v_nominal_specify=off  v_nominal_value=1  v_nominal_unit=V
  Diode2 : fl_lib/Electrical/Electrical Elements/Diode  Commented=on  Vf=0.6 V  Ron=0.3 Ohm  Goff=1e-8 1/Ohm  i_specify=off  i_priority=None  i=0 A  i_nominal_specify=off  i_nominal_value=1  i_nominal_unit=A  v_specify=off  v_priority=None  v=0 V  v_nominal_specify=off  v_nominal_value=1  v_nominal_unit=V
  Diode3 : fl_lib/Electrical/Electrical Elements/Diode  Commented=on  Vf=0.6 V  Ron=0.3 Ohm  Goff=1e-8 1/Ohm  i_specify=off  i_priority=None  i=0 A  i_nominal_specify=off  i_nominal_value=1  i_nominal_unit=A  v_specify=off  v_priority=None  v=0 V  v_nominal_specify=off  v_nominal_value=1  v_nominal_unit=V
  Electrical Reference3 : fl_lib/Electrical/Electrical Elements/Electrical Reference  Commented=on
  Electrical Reference4 : fl_lib/Electrical/Electrical Elements/Electrical Reference  Commented=on
  Electrical Reference5 : fl_lib/Electrical/Electrical Elements/Electrical Reference  Commented=on
  "IGBT (Ideal, Switching)" : ee_lib/Semiconductors & Converters/IGBT (Ideal, Switching)  Commented=on  port_option=ee.enum.controlport.elec  Vf=0.8 V  Ron=0.001 Ohm  Goff=1e-5 1/Ohm  Vth=2 V  diode_param=1  diode_Vf=0.8 V  diode_Ron=0.001 Ohm  diode_Goff=1e-5 1/Ohm  diode_C=50e-9 F  diode_iRM=-235 A  diode_iF=300 A  diode_idot=-50 A/us  diode_trr_param=1  diode_trr_factor=3  diode_trr=15 us  diode_Qrr=1500 s*uA  ice_specify=off  ice_priority=None  ice=0 A  ice_nominal_specify=off  ice_nominal_value=1  ice_nominal_unit=A  vce_specify=off  vce_priority=None  vce=0 V  vce_nominal_specify=off  vce_nominal_value=1  vce_nominal_unit=V  vge_specify=off  vge_priority=None  vge=0 V  vge_nominal_specify=off  vge_nominal_value=1  vge_nominal_unit=V  thermal_loss_option=2  Von_data=[0, 1.1, 1.3, 1.45, 1.75, 2.25, 2.7; 0, 1, 1.15, 1.35, 1.7, 2.35, 3] V  Tj=[298.15, 398.15] K  Iout_data=[0, 10, 50, 100, 200, 400, 600] A  Eon_data=[0, .29, 1.43, 2.86, 5.71, 13.14, 22.86; 0, .57, 2.63, 5.14, 10.29, 20.57, 30.29] * 1e-3 J  Eoff_data=[0, .21, 1.07, 2.14, 4.29, 9.86, 17.14; 0, .43, 1.97, 3.86, 7.71, 15.43, 22.71] * 1e-3 J  Eon_data_3D=[zeros(2, 9, 3)] J  Eoff_data_3D=[zeros(2, 9, 3)] J  Tj_loss=[298.15, 398.15] K  Iout_data_loss=[0, .1, 1, 5, 10, 20, 40, 70, 100] A  tabulateWithVce=false  Vce_loss=[0, 150, 300] V  Eon_scalar=22.86e-3 J  Eoff_scalar=17.14e-3 J  Voff=300 V  Iout_scalar=600 A  useCurrentFromPreviousCycle=false  useVoltageFromPreviousCycle=false  diodeModelType=ee.enum.converters.diodeModelType.pwl  diodeTableType=ee.enum.diode.tableType.IfMat  diode_ReverseIVType=ee.enum.diode.diodeReverseIV.constant  diode_IfMat=[.07, .12, .19, 1.75, 4.24, 7.32, 11.2; .16, .3, .72, 2.14, 4.02, 6.35, 9.12] A  diode_VfMat=[.9, 1.15, 1.25, 1.5, 1.75, 2.17, 2.6, 2.85; .58, .68, .75, 1.1, 1.38, 1.77, 2.27, 2.7] V  diode_TjVec=[25, 125] degC  diode_VfVec=[.5, .7, .9, 1.3, 1.7, 2.1, 2.5] V  diode_IfVec=[.1, .2, .5, 1, 2, 4, 7, 10] A  diode_IrMat=[1e-06, 2e-06, 5e-06, 1e-05, 2.5e-05, 5e-05, .0001; 2e-06, 5e-06, 1e-05, 4e-05, 8e-05, .0002, .0005] A  diode_VrMat=[10, 100, 200, 250, 300, 325, 350; 10, 70, 160, 220, 270, 300, 320] V  diode_VrVec=[10, 20, 40, 50, 70, 80, 100] V  diode_IrVec=[1e-06, 2e-06, 5e-06, 1e-05, 2e-05, 5e-05, .0001] A  diode_Vr=-600 V  diode_Ls=150 nH  diode_Erec=0.03 J  diode_rec_loss_model=ee.enum.diode.reverseRecoveryModel.fixed  diode_ErecVal=0 J  diode_scaleWithIandV=true  diode_ErecMat=zeros(2, 3) J  diode_TjrecVec=[298.15, 398.15] K  diode_IfrecVec=[.1, 1, 10] A  diode_IrecVal=10 A  diode_VrecVal=10 V  diode_tFilter=1 / 1000 / 100 s  separateThermalPortForDiode=false  thermal_network_parameterization=ee.enum.thermalNetworkTopology.external  Rth=[.08, .5] K/W  Rth_Cauer=[.08, .1, .5] K/W  Rth_Foster=[.08, .14, .22, .16] K/W  thermal_mass_parameterization=ee.enum.thermalNetwork.timeconstant  thermal_mass=[.01, .5] J/K  thermal_mass_Cauer=[.01, .1, .5] J/K  thermal_mass_Foster=[.001, .005, .05, .5] J/K  thermal_time_constant=[.001, .2] s  thermal_time_constant_Cauer=[.001, .1, .2] s  thermal_time_constant_Foster=[7e-05, .0007, .01, .08] s  thermal_mass_initial_temperatures=[25, 25] degC  thermal_mass_initial_temperatures_Cauer=[25, 25, 25] degC  junction_thermal_mass=0.01 J/K  Tvec_initial_Foster=[25, 25, 25, 25] degC  RthDiode=[.03, .2] K/W  RthCauerDiode=[.03, .1, .2] K/W  RthFosterDiode=[.03, .2] K/W  thermalMassDiode=[3, 25] J/K  thermalMassCauerDiode=[3, 10, 25] J/K  thermalMassFosterDiode=[33, 50] J/K  thermalTauDiode=[.1, 5] s  thermalTauCauerDiode=[.1, 1, 5] s  thermalTauFosterDiode=[1, 10] s  thermalMassInitTempDiode=[25, 25] degC  thermalMassInitTempCauerDiode=[25, 25, 25] degC  junctionthermalMassDiode=0.1 J/K  TVecInitialFosterDiode=[25, 25, 25, 25] degC  no_thermal_network=0  IGBT_junction_temperature_specify=off  IGBT_junction_temperature_priority=None  IGBT_junction_temperature=25 degC  IGBT_junction_temperature_nominal_specify=off  IGBT_junction_temperature_nominal_value=1  IGBT_junction_temperature_nominal_unit=degC  diode_junction_temperature_specify=off  diode_junction_temperature_priority=None  diode_junction_temperature=25 degC  diode_junction_temperature_nominal_specify=off  diode_junction_temperature_nominal_value=1  diode_junction_temperature_nominal_unit=degC  Qj_specify=off  Qj_priority=None  Qj=0 W  Qj_nominal_specify=off  Qj_nominal_value=1  Qj_nominal_unit=W  accumulatedSwitchingLosses_specify=off  accumulatedSwitchingLosses_priority=None  accumulatedSwitchingLosses=0 J
      settings: InternalSimscapePortConfiguration="{\"Bottom\":[],\"Left\":[{\"id\":\"G_elec\",\"label\":\"\",\"type\":\"foundation.electrical.electrical\"}],\"Right\":[{\"id\":\"C\",\"label\":\"\",\"type\":\"foundation.electrical.electrical\"},{\"id\":\"E\",\"label\":\"\",\"type\":\"foundation.electrical.electrical\"}],\"Top\":[]}"
  Ideal Transformer : fl_lib/Electrical/Electrical Elements/Ideal Transformer  Commented=on  n=2  i1_specify=off  i1_priority=None  i1=0 A  i1_nominal_specify=off  i1_nominal_value=1  i1_nominal_unit=A  v1_specify=off  v1_priority=None  v1=0 V  v1_nominal_specify=off  v1_nominal_value=1  v1_nominal_unit=V  i2_specify=off  i2_priority=None  i2=0 A  i2_nominal_specify=off  i2_nominal_value=1  i2_nominal_unit=A  v2_specify=off  v2_priority=None  v2=0 V  v2_nominal_specify=off  v2_nominal_value=1  v2_nominal_unit=V
  PS Constant : fl_lib/Physical Signals/Sources/PS Constant  Commented=on  constant=48 V
  Resistor1 : fl_lib/Electrical/Electrical Elements/Resistor  Commented=on  R=470 Ohm  i_specify=off  i_priority=None  i=0 A  i_nominal_specify=off  i_nominal_value=1  i_nominal_unit=A  v_specify=off  v_priority=None  v=0 V  v_nominal_specify=off  v_nominal_value=1  v_nominal_unit=V
  Resistor3 : fl_lib/Electrical/Electrical Elements/Resistor  Commented=on  R=470 Ohm  i_specify=off  i_priority=None  i=0 A  i_nominal_specify=off  i_nominal_value=1  i_nominal_unit=A  v_specify=off  v_priority=None  v=0 V  v_nominal_specify=off  v_nominal_value=1  v_nominal_unit=V
  Resistor5 : fl_lib/Electrical/Electrical Elements/Resistor  Commented=on  R=100 Ohm  i_specify=off  i_priority=None  i=0 A  i_nominal_specify=off  i_nominal_value=1  i_nominal_unit=A  v_specify=off  v_priority=None  v=0 V  v_nominal_specify=off  v_nominal_value=1  v_nominal_unit=V
  Resistor6 : fl_lib/Electrical/Electrical Elements/Resistor  Commented=on  R=1e9 Ohm  i_specify=off  i_priority=None  i=0 A  i_nominal_specify=off  i_nominal_value=1  i_nominal_unit=A  v_specify=off  v_priority=None  v=0 V  v_nominal_specify=off  v_nominal_value=1  v_nominal_unit=V
  Voltage Sensor : fl_lib/Electrical/Electrical Sensors/Voltage Sensor  Commented=on
  oscillator : Subsystem  Commented=on
  gin : PMIOPort  Side=Left
  g+ : PMIOPort  Port=2  Side=Right
  connections:
  Resistor3/LConn1 -- Controlled Voltage Source1/LConn1
  Electrical Reference5/LConn1 -- Capacitor1/RConn1
  Capacitor1/LConn1 -- Resistor3/RConn1 -- Diode3/LConn1
  "IGBT (Ideal, Switching)"/RConn1 -- Diode3/RConn1
  Resistor6/RConn1 -- Electrical Reference3/LConn1
  PS Constant/RConn1 -- Controlled Voltage Source1/RConn1
  Capacitor2/LConn1 -- Voltage Sensor/LConn1 -- Resistor5/LConn1 -- Diode2/RConn1
  Resistor5/RConn1 -- Resistor6/LConn1 -- Ideal Transformer/RConn2 -- Voltage Sensor/RConn2 -- Capacitor2/RConn1
  Ideal Transformer/RConn1 -- Diode2/LConn1
  Diode/RConn1 -- Ideal Transformer/LConn1 -- "IGBT (Ideal, Switching)"/RConn2 -- Controlled Voltage Source1/RConn2 -- Controlled Voltage Source2/RConn2
  Controlled Voltage Source2/LConn1 -- Resistor1/LConn1
  Ideal Transformer/LConn2 -- Diode/LConn1 -- Electrical Reference4/LConn1
  "IGBT (Ideal, Switching)"/LConn1 -- Resistor1/RConn1
  gin/RConn1 -- g+/RConn1
